simulink model "lab"  (R2023a)
settings: Solver=FixedStepDiscrete  StartTime=0.0  StopTime=inf  RelTol=1e-3  EnableMultiTasking=on
PreLoadFcn:
  | gCSP_Precursor_OFF=Simulink.Variant('gCSP_Precursor==0');
  | gCSP_Precursor_ON=Simulink.Variant('gCSP_Precursor==1');
  | 
  | gCSP_Precursor=0;
InitFcn:
  | global FeedbackGain;
  | FeedbackGain = 0.1;
  | 
  | if exist('WV') ~= 1
  | global WV
  | WV = zeros(1, 5);
  | end
  | 
  | NumberOfChannels = MultiDeviceDAQ_getNumChannels;
  | if (exist('W_CSP') ~= 1)
  |     global W_CSP
  |     if NumberOfChannels == 63
  |         try
  |            SPF = spf;
  |            Filter=load(SPF,'generic_CSP_2Class_63channels.mat');
  |            sf = get(Filter,'spf');
  |            spf_struct = struct(sf);
  |            W_CSP = spf_struct.D.W;
  |         catch
  |             W_CSP = zeros(NumberOfChannels,NumberOfChannels);
  |         end
  |     elseif NumberOfChannels == 27
  |         try
  |             W_CSPt = load('template_W_CSP_TwoClasses_27Ch');
  |             W_CSP = W_CSPt.W_CSP;
  |         catch
  |             W_CSP = zeros(NumberOfChannels,NumberOfChannels);
  |         end
  | elseif NumberOfChannels == 16
  |         try
  |             W_CSPt = load('template_W_CSP_TwoClasses_16Ch');
  |             W_CSP = W_CSPt.W_CSP;
  |         catch
  |             W_CSP = zeros(NumberOfChannels,NumberOfChannels);
  |         end
  |     else
  |         W_CSP = zeros(NumberOfChannels,NumberOfChannels);
  |     end
  | end
StartFcn:
  | NumberOfChannels = MultiDeviceDAQ_getNumChannels;
  | 
  | NumCsps = size(W_CSP,1);
  | 
  | if (NumCsps ~= NumberOfChannels)
  | troubles('The number of selected channels does not fit to the number of channels used for setting up the CSPs',['Select the channels in the Select Channels -block to get ',num2str(NumCsps),' channels. If you have changed the electrode configuration please restart Matlab.']);
  | set_param(gcs, 'SimulationCommand', 'stop');
  | end
values from neighbouring files (symbols this model uses):
  spf = get(Filter,'spf')    [CreateClassifier_CSP_TwoClass.m]
undefined symbols (not defined in the file or in its folder): MultiDeviceDAQ_getSampleRate
libraries: FeatureExtraction x4, Classification x1, Preprocessing x1, gSTIMboxlib x1, DataStream x1, Visualization x1, DataAcquisition x1
CloseFcn:
  | clear W_CSP;
Description:
  | g.USBamp based CSP MI BCI for two classes
  | 
  | Copyright g.tec medical engineering GmbH
settings Model: ModifiedByFormat=g.tec  Creator=circuit  LastModifiedBy=g.tec
settings SolverCC: AlgebraicLoopSolver=TrustRegion
settings DataIOCC: LimitDataPoints=on  SaveFormat=Array  SignalLoggingSaveFormat=ModelDataLogs  ReturnWorkspaceOutputs=off
settings OptimizationCC: BlockReduction=off  ExpressionDepthLimit=2147483647  InitFltsAndDblsToZero=on  LifeSpan=inf
settings DebuggingCC: SaveWithParameterizedLinksMsg=none  UnderspecifiedInitializationDetection=Classic  MergeDetectMultiDrivingBlocksExec=none  SolverPrmCheckMsg=warning  FcnCallInpInsideContextMsg=warning  UnconnectedInputMsg=warning  UnconnectedOutputMsg=warning  UnconnectedLineMsg=warning  StateNameClashWarn=warning  SFUnexpectedBacktrackingDiag=warning  SFNoUnconditionalDefaultTransitionDiag=warning  SFExecutionAtInitializationDiag=none  ArithmeticOperatorsInVariantConditions=warning
settings HardwareCC: ProdBitPerPointer=32  ProdBitPerSizeT=32  ProdBitPerPtrDiffT=32  ProdLargestAtomicFloat=None  ProdIntDivRoundTo=Undefined  ProdEndianess=Unspecified  ProdWordSize=32  ProdHWDeviceType=32-bit Generic
settings ModelReferenceCC: EnableRefExpFcnMdlSchedulingChecks=on  PropagateSignalLabelsOutOfModel=off
settings SFSimCC: SimUseLocalCustomCode=off  CustomCodeUndefinedFunction=UseInterfaceOnly
settings RTWCC: RTWUseLocalCustomCode=off
settings CodeAppCC: StateflowObjectComments=on
settings GRTTargetCC: TargetLangStandard=C89/C90 (ANSI)  CombineOutputUpdateFcns=off  GRTInterface=on
settings ConfigComp: CovMetricSettings=dw  CovSaveCumulativeToWorkspaceVar=on  CovSaveSingleToWorkspaceVar=on  CovExternalEMLEnable=off  CovSFcnEnable=off

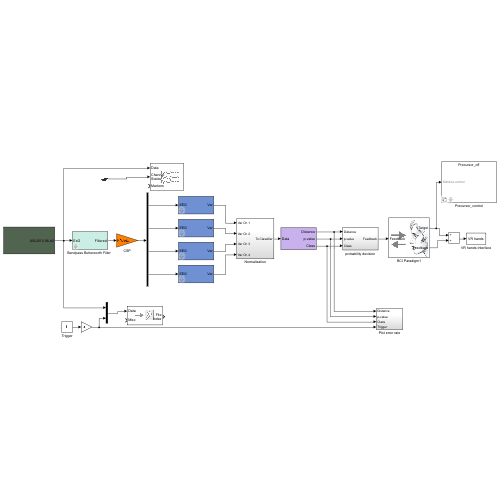
[thumbnail: Simulink's stored preview of the top-level diagram]
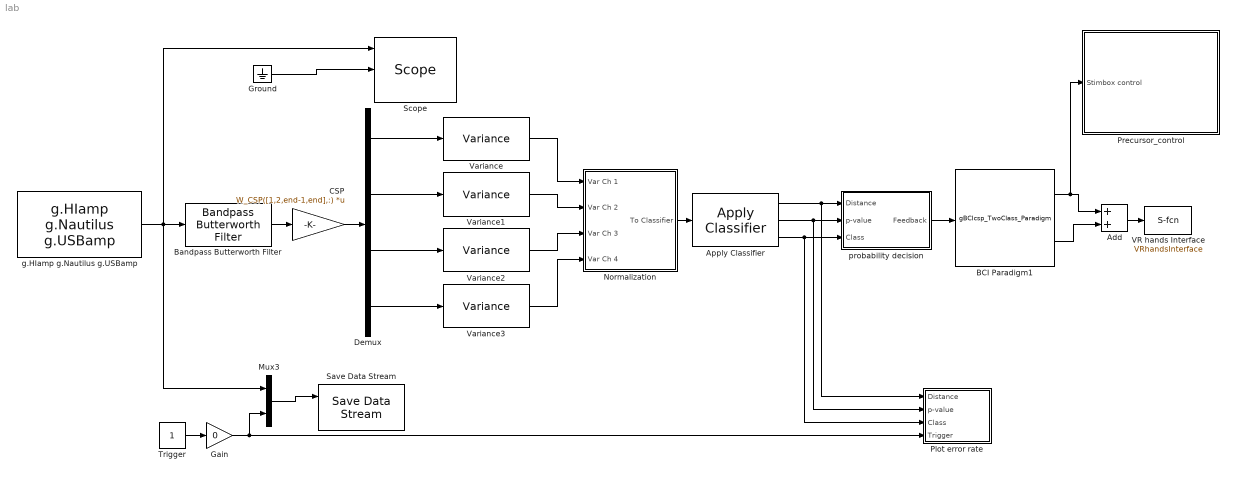
== system lab ==
  Add : Sum
  Apply Classifier : Classification/Apply Classifier
      settings: SourceProductName=g.HIsys
  BCI Paradigm1 : M-S-Function  FunctionName=gBCIcsp_TwoClass_Paradigm  Parameters=paradigm, runnumber, MultiDeviceDAQ_getSampleRate  mask(BCI Paradigm Block){paradigm=feedback, runnumber=4, precursor=off}
      mask prompts: runnumber "Run number:"; precursor "Tactile pre cursor"
      mask TypeOptions paradigm: no feedback | feedback | ball
      mask TypeOptions runnumber: 1 | 2 | 3 | 4
      mask Display:
      | image(imread('feedback_symb.tif'))
      | port_label('output', 1, 'Target');
      | port_label('output', 2, 'Feedback');
      | port_label('input', 1, 'Feedback');
  "Bandpass Butterworth Filter  " : Preprocessing/Bandpass Butterworth Filter  LPOrder=5  UpperFreq=30  HPOrder=5  LowerFreq=8  SampFreq=MultiDeviceDAQ_getSampleRate
      settings: SourceProductName=g.HIsys
  CSP : Gain  Gain=W_CSP([1,2,end-1,end],:)  Multiplication=Matrix(K*u) (u vector)
  Demux : Demux
  Gain : Gain  Gain=0
  Ground : Ground
  Mux3 : Mux  Inputs=2
  Normalization : Subsystem
  Plot error rate : Subsystem  Priority=3
  Precursor_control : Subsystem  Variant=on  mask{PrecursorRadiobutton=Off}
      mask prompts: PrecursorRadiobutton "Tactile pre-cursor"
      mask help: Use this mask to enable or disable the tactile pre-cursor.
      mask Help: See the manual for help.
      mask TypeOptions PrecursorRadiobutton: On | Off
      mask Callback PrecursorRadiobutton:
      | radiobuttonStatus = get_param([gcs,'/Precursor_control'],'PrecursorRadioButton');
      | maskHandle = Simulink.Mask.get(gcb);
      | StimboxButtonHandle = maskHandle.getDialogControl('openStimboxUI');
      | 
      | if strcmp(radiobuttonStatus,'On')
      |     gCSP_Precursor = 1;
      |     StimboxButtonHandle.Enabled = 'on';
      | %     disp('on');
      | elseif strcmp(radiobuttonStatus,'Off')
      |     gCSP_Precursor = 0;
      |     StimboxButtonHandle.Enabled = 'off';
      | 
      | %     disp('off');
      | end
      mask DialogControl openStimboxUI Prompt: open the g.STIMbox interface
      mask DialogControl openStimboxUI Callback:
      | % open the stimbox UI to enter the COM port
      |     stimboxBlockHandle = get_param([get_param(gcs,'Name'),'/Precursor_control/Precursor_on/STIMbox'],'Handle');
      |     gSTIMboxGUI_openDlg('STIMboxGUI', stimboxBlockHandle);
  Save Data Stream : DataStream/Save Data Stream  filename=Exp_1_Run_4.mat  filesize=100  blocksize=512  rec_type=Double  enable=off  save_model=off  save_pp_taskinfo=off  patient_data=off  id=ID0000  firstname=John  lastname=Doe  dateofbirth=12.01.2001  sex=MALE  hand=RIGHT  diagnosis=Diagnosis  medication=Medication Text  comments=any text ...  run=1  session=1
      settings: SourceProductName=g.HIsys
  Scope : Visualization/Scope
      settings: SourceProductName=g.HIsys
  Trigger : Constant  SampleTime=1/MultiDeviceDAQ_getSampleRate
  VR hands Interface : M-S-Function  FunctionName=VRhandsInterface  Parameters=IP,VRhands  mask(VR hands interface){VRhands=off, IP=192.168.0.1}
      mask prompts: VRhands "Use VRhands interface"
      mask Callback VRhands:
      | if (strcmp(get_param(gcb,'VRhands'),'on'))
      | set_param(gcb,'MaskEnables',{'on';'on'});
      | elseif (strcmp(get_param(gcb,'VRhands'),'off'))
      | set_param(gcb,'MaskEnables',{'on';'off'});
      | end
      mask Callback IP:
      | IP = get_param(gcb,'IP');
      | if isempty(IP)
      |     IP = '192.168.0.1'; set_param(gcb,'IP',IP);
      | else
      |     IP4 = regexp(IP, '\W', 'split'); IP_chk = zeros(1,4);
      |     if size(IP4,2) == 4
      |         for ii = 1:4
      |             IP_temp = str2num(IP4{ii});
      |             if isempty(IP_temp)
      |                 IP_temp = 0;
      |             else
      |                 if size(IP_temp)~=[1,1]
      |                     IP_temp = IP_temp(1,1);
      |                 end
      |                 if IP_temp<0
      |                     IP_temp = abs(IP_temp);
      |                 end
      |                 if IP_temp>255
      |                     IP_temp = 255;
      |                 end
      |             end
      |             IP_chk(ii)=IP_temp;
      |         end
      |         IP = [num2str(IP_chk(1)),'.',num2str(IP_chk(2)),'.',num2str(IP_chk(3)),'.',num2str(IP_chk(4))];set_param(gcb,'IP',IP);
      |     else
      |         IP = '192.168.0.1';set_param(gcb,'IP',IP);
      |     end
      | end
      | clear IP IP4 IP_chk IP_temp ii;
      mask Display: disp('VR hands')
  Variance{,1..3} (4 alike) : FeatureExtraction/Variance  WindowLength=384
      settings: SourceProductName=g.HIsys
  g.HIamp g.Nautilus g.USBamp : DataAcquisition/g.HIamp g.Nautilus g.USBamp  cfgUpdated=739941.4956  numDevices=2  deviceSR=[500 250 ]  deviceChannels=[9 4 ]  numSR=[2 ]  SRIndexPerDevice=[1 0 ]
      settings: SourceProductName=g.HIsys
  probability decision : Subsystem
  wires:
  Demux/1 -> Variance/1
  Demux/3 -> Variance2/1
  Demux/4 -> Variance3/1
  Demux/2 -> Variance1/1
  Variance/1 -> Normalization/1(Var Ch 1)
  Variance2/1 -> Normalization/3(Var Ch 3)
  Variance3/1 -> Normalization/4(Var Ch 4)
  Mux3/1 -> Save Data Stream/1
  Normalization/1(To Classifier) -> Apply Classifier/1
  Variance1/1 -> Normalization/2(Var Ch 2)
  Trigger/1 -> Gain/1
  Gain/1 -> Mux3/2, Plot error rate/4(Trigger)
  Apply Classifier/2 -> Plot error rate/2(p-value), probability decision/2(p-value)
  Apply Classifier/3 -> Plot error rate/3(Class), probability decision/3(Class)
  Apply Classifier/1 -> Plot error rate/1(Distance), probability decision/1(Distance)
  probability decision/1(Feedback) -> BCI Paradigm1/1
  g.HIamp g.Nautilus g.USBamp/1 -> "Bandpass Butterworth Filter  "/1, Scope/1, Mux3/1
  Add/1 -> VR hands Interface/1
  BCI Paradigm1/1 -> Precursor_control/1(Stimbox control), Add/1
  BCI Paradigm1/2 -> Add/2
  Ground/1 -> Scope/2
  "Bandpass Butterworth Filter  "/1 -> CSP/1
  CSP/1 -> Demux/1

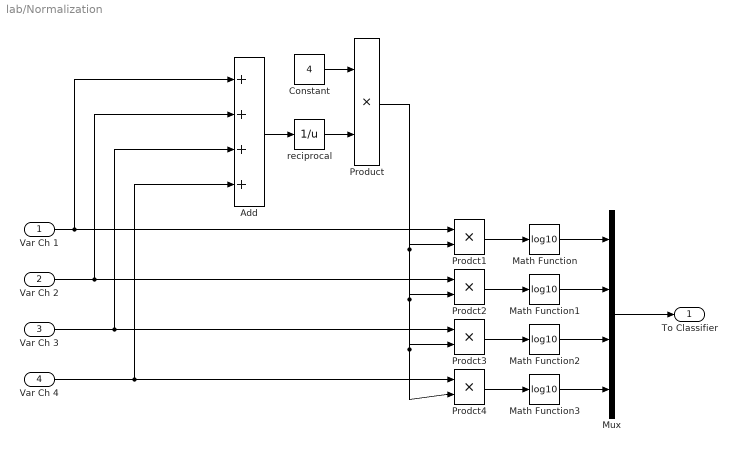
== system lab/Normalization ==
  Var Ch 1 : Inport
  Var Ch 2 : Inport  Port=2
  Var Ch 3 : Inport  Port=3
  Var Ch 4 : Inport  Port=4
  Add : Sum  Inputs=++++
  Constant : Constant  Value=4
  Math Function{,1..3} (4 alike) : Math  Operator=log10  SignedPower=on
  Mux : Mux
  Prodct{1..4} (4 alike) : Product  RndMeth=Zero
  Product : Product  RndMeth=Zero
  reciprocal : Math  Operator=reciprocal  SignedPower=on
  To Classifier : Outport
  wires:
  Var Ch 1/1 -> Add/1, Prodct1/1
  Var Ch 3/1 -> Add/3, Prodct3/1
  Var Ch 4/1 -> Add/4, Prodct4/1
  Constant/1 -> Product/1
  reciprocal/1 -> Product/2
  Var Ch 2/1 -> Add/2, Prodct2/1
  Add/1 -> reciprocal/1
  Prodct1/1 -> Math Function/1
  Prodct2/1 -> Math Function1/1
  Prodct3/1 -> Math Function2/1
  Prodct4/1 -> Math Function3/1
  Product/1 -> Prodct4/2, Prodct3/2, Prodct2/2, Prodct1/2
  Math Function/1 -> Mux/1
  Math Function1/1 -> Mux/2
  Math Function2/1 -> Mux/3
  Math Function3/1 -> Mux/4
  Mux/1 -> To Classifier/1

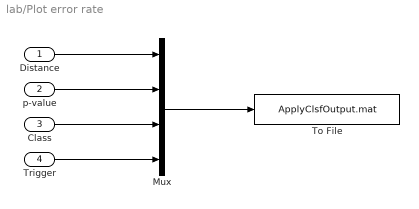
== system lab/Plot error rate ==
  Distance : Inport
  p-value : Inport  Port=2
  Class : Inport  Port=3
  Trigger : Inport  Port=4
  Mux : Mux
  To File : ToFile  Filename=ApplyClsfOutput.mat  MatrixName=y
  wires:
  Distance/1 -> Mux/1
  p-value/1 -> Mux/2
  Class/1 -> Mux/3
  Trigger/1 -> Mux/4
  Mux/1 -> To File/1

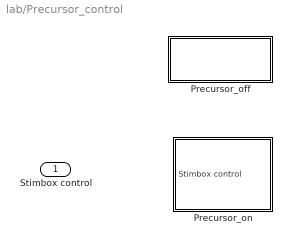
== system lab/Precursor_control ==
  Stimbox control : Inport
  Precursor_off : Subsystem  VariantControl=gCSP_Precursor_OFF
  Precursor_on : Subsystem  VariantControl=gCSP_Precursor_ON

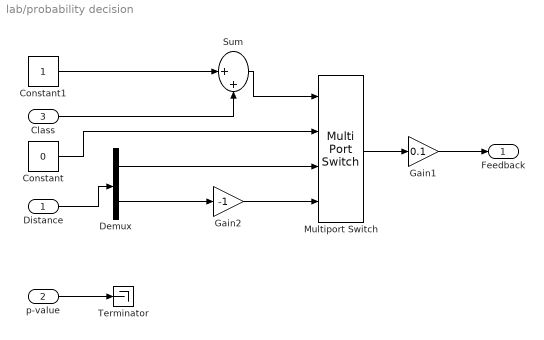
== system lab/probability decision ==
  Distance : Inport
  p-value : Inport  Port=2
  Class : Inport  Port=3
  Constant : Constant  Value=0
  Constant1 : Constant
  Demux : Demux  Outputs=2
  Gain1 : Gain  Gain=0.1
  Gain2 : Gain  Gain=-1
  Multiport Switch : MultiPortSwitch  SaturateOnIntegerOverflow=off  InputSameDT=off
  Sum : Sum  Inputs=|++
  Terminator : Terminator
  Feedback : Outport
  wires:
  Gain1/1 -> Feedback/1
  Distance/1 -> Demux/1
  Demux/2 -> Gain2/1
  Multiport Switch/1 -> Gain1/1
  Sum/1 -> Multiport Switch/1
  Gain2/1 -> Multiport Switch/4
  Demux/1 -> Multiport Switch/3
  Constant/1 -> Multiport Switch/2
  p-value/1 -> Terminator/1
  Class/1 -> Sum/2
  Constant1/1 -> Sum/1

== system lab/Precursor_control/Precursor_off ==

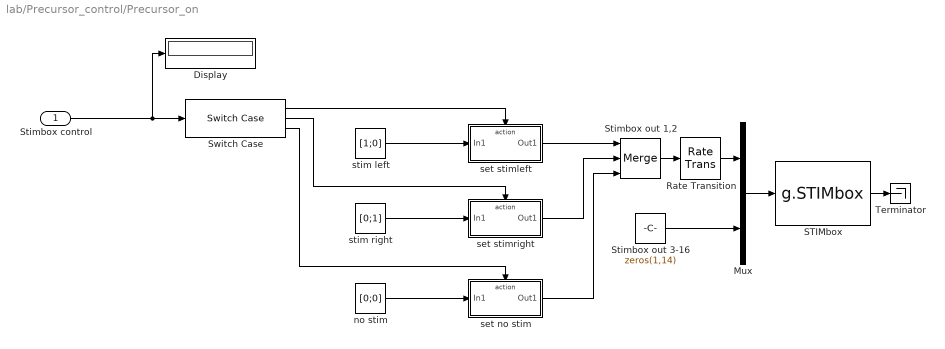
== system lab/Precursor_control/Precursor_on ==
  Stimbox control : Inport
  Display : Display
  Mux : Mux  Inputs=2
  Rate Transition : RateTransition
  STIMbox : gSTIMboxlib/g.STIMbox  comport=4  sr=64  fl=1  ia=1  bm=1  fs=1  chmodes="[0  0  0  0  0  0  0  0  0  0  0  0  0  0  0  0]"  chfreqs="[1  1  1  1  1  1  1  1  1  1  1  1  1  1  1  1]"  chinv="[0  0  0  0  0  0  0  0  0  0  0  0  0  0]"
  Stimbox out 1,2 : Merge  Inputs=3
  Stimbox out 3-16 : Constant  Value=zeros(1,14)  SampleTime=1/64
  Switch Case : SwitchCase  CaseConditions={-1,1,0}  ShowDefaultCase=off
  Terminator : Terminator
  no stim : Constant  Value=[0;0]
  set no stim : Subsystem  TreatAsAtomicUnit=on
  set stimleft : Subsystem  TreatAsAtomicUnit=on
  set stimright : Subsystem  TreatAsAtomicUnit=on
  stim left : Constant  Value=[1;0]
  stim right : Constant  Value=[0;1]
  wires:
  Switch Case/1 -> set stimleft/Action
  Switch Case/2 -> set stimright/Action
  Switch Case/3 -> set no stim/Action
  Stimbox control/1 -> Display/1, Switch Case/1
  stim left/1 -> set stimleft/1(In1)
  stim right/1 -> set stimright/1(In1)
  no stim/1 -> set no stim/1(In1)
  set stimleft/1(Out1) -> Stimbox out 1,2/1
  set stimright/1(Out1) -> Stimbox out 1,2/2
  set no stim/1(Out1) -> Stimbox out 1,2/3
  Stimbox out 3-16/1 -> Mux/2
  Mux/1 -> STIMbox/1
  STIMbox/1 -> Terminator/1
  Stimbox out 1,2/1 -> Rate Transition/1
  Rate Transition/1 -> Mux/1

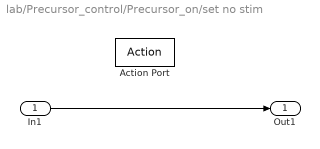
== system lab/Precursor_control/Precursor_on/set no stim ==
  In1 : Inport
  Action Port : ActionPort
  Out1 : Outport
  wires:
  In1/1 -> Out1/1

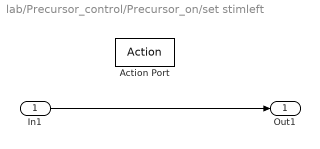
== system lab/Precursor_control/Precursor_on/set stimleft ==
  In1 : Inport
  Action Port : ActionPort
  Out1 : Outport
  wires:
  In1/1 -> Out1/1

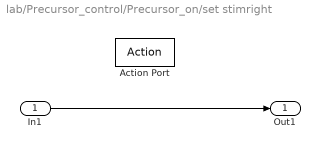
== system lab/Precursor_control/Precursor_on/set stimright ==
  In1 : Inport
  Action Port : ActionPort
  Out1 : Outport
  wires:
  In1/1 -> Out1/1
